simulink model "all_at_0001_0101"  (R2026a)
settings: Solver=ode5  StopTime=30  FixedStep=.01  AbsTol=1e-6
model workspace (MATLAB code in the model file):
  | load sldemo_autotrans_data; %load initial conditions and other necessary data
undefined symbols (not defined in the file): converter_data, downtab, emap, Iei, uptab, vehicledata
Description:
  | Modeling an Automatic Transmission Controller
  | 
  | In this example, Simulink(R) is used to model an automotive drivetrain. Stateflow(R)
  | enhances the Simulink model with its representation of the transmission
  | control logic. Simulink provides a powerful environment for the modeling and
  | simulation of dynamic systems and processes. In many systems, though,
  | supervisory functions like changing modes or invoking new gain schedules must
  | respond to events that may occur and conditions that develop over time. As a
  | result, the environment requires a language capable of managing these multiple
  | modes and developing conditions. In the following example, Stateflow
  | demonstrates its strength in this capacity by performing the function of gear
  | selection in an automatic transmission. This function is combined with the
  | drivetrain dynamics in a natural and intuitive manner by incorporating a
  | Stateflow block in the Simulink block diagram.
settings Model: DataTypeOverride=Double  MinMaxOverflowLogging=ForceOff  SimulationMode=accelerator  ExtModeTrigMode=oneshot  ExtModeArmWhenConnect=off  ExtModeAutoUpdateStatusClock=off  Creator=The MathWorks Inc.  LastModifiedBy=harry_31916
settings DataIOCC: ExternalInput=[t__, u__]  SignalLoggingName=sldemo_autotrans_output
settings OptimizationCC: BooleanDataType=off  InitFltsAndDblsToZero=on
settings DebuggingCC: SaveWithParameterizedLinksMsg=none  UnderspecifiedInitializationDetection=Classic  CheckExecutionContextPreStartOutputMsg=on  SignalResolutionControl=TryResolveAllWithWarning  MultiTaskDSMMsg=warning  MultiTaskCondExecSysMsg=none  SigSpecEnsureSampleTimeMsg=none  IntegerOverflowMsg=none  IntegerSaturationMsg=none
settings HardwareCC: ProdHWDeviceType=32-bit Generic
settings SFSimCC: SFSimEcho=off
settings GRTTargetCC: TargetFcnLib=ansi_tfl_tmw.mat  CombineOutputUpdateFcns=off  GRTInterface=on
settings ConfigComp: CovMetricSettings=dcmtr

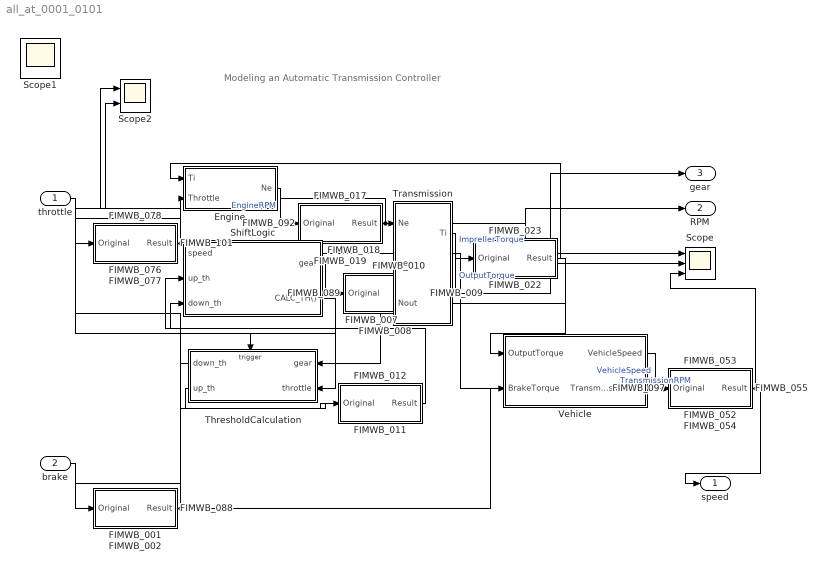
== system all_at_0001_0101 ==
  note: Modeling an Automatic Transmission Controller
  throttle : Inport  Interpolate=off
  brake : Inport  Port=2  Interpolate=off
  Engine : Subsystem
  FIMWB_001 : Subsystem  Tag=fimwb.fault.1
  FIMWB_002 : Subsystem  Tag=fimwb.fault.2
  FIMWB_007 : Subsystem  Tag=fimwb.fault.7
  FIMWB_008 : Subsystem  Tag=fimwb.fault.8
  FIMWB_009 : Subsystem  Tag=fimwb.fault.9
  FIMWB_010 : Subsystem  Tag=fimwb.fault.10
  FIMWB_011 : Subsystem  Tag=fimwb.fault.11
  FIMWB_012 : Subsystem  Tag=fimwb.fault.12
  FIMWB_017 : Subsystem  Tag=fimwb.fault.17
  FIMWB_018 : Subsystem  Tag=fimwb.fault.18
  FIMWB_019 : Subsystem  Tag=fimwb.fault.19
  FIMWB_022 : Subsystem  Tag=fimwb.fault.22
  FIMWB_023 : Subsystem  Tag=fimwb.fault.23
  FIMWB_052 : Subsystem  Tag=fimwb.fault.52
  FIMWB_053 : Subsystem  Tag=fimwb.fault.53
  FIMWB_054 : Subsystem  Tag=fimwb.fault.54
  FIMWB_055 : Subsystem  Tag=fimwb.fault.55
  FIMWB_076 : Subsystem  Tag=fimwb.fault.76
  FIMWB_077 : Subsystem  Tag=fimwb.fault.77
  FIMWB_078 : Subsystem  Tag=fimwb.fault.78
  FIMWB_088 : Subsystem  Tag=fimwb.fault.88
  FIMWB_089 : Subsystem  Tag=fimwb.fault.89
  FIMWB_092 : Subsystem  Tag=fimwb.fault.92
  FIMWB_097 : Subsystem  Tag=fimwb.fault.97
  FIMWB_101 : Subsystem  Tag=fimwb.fault.101
  Scope : Scope  NumInputPorts=3
      settings: ActiveDisplayYMinimum=-5  ActiveDisplayYMaximum=5
  Scope2 : Scope  NumInputPorts=2
      settings: ActiveDisplayYMinimum=-5  ActiveDisplayYMaximum=100
  ShiftLogic : Stateflow chart  TreatAsAtomicUnit=on
  ThresholdCalculation : Subsystem  TreatAsAtomicUnit=on
  Transmission : Subsystem
  Vehicle : Subsystem  mask(vehicle model){Rfd=vehicledata(1), rload0=vehicledata(2), rload2=vehicledata(3), Rw=vehicledata(4), Iv=vehicledata(5), N20=vehicledata(6)/vehicledata(4)*vehicledata(1)}
      mask prompts: Rfd "final drive ratio"; rload0 "drag friction at wheels"; rload2 "aerodynamic drag"; Rw "wheel radius"; Iv "vehicle inertia"; N20 "initial transmission output speed"
      mask help: vehicle dynamics: torque input from trans., outputs are input speed (transmission output) and vehicle speed
      mask Display: image(imread([matlabroot,'/toolbox/simulink/simdemos/automotive/html/NSX_3Colors.jpg']))
  speed : Outport  VectorParamsAs1DForOutWhenUnconnected=off
  RPM : Outport  Port=2  VectorParamsAs1DForOutWhenUnconnected=off
  gear : Outport  Port=3  VectorParamsAs1DForOutWhenUnconnected=off
  Scope1 : Scope
      settings: TimeSpan=30  ActiveDisplayYMinimum=1000  ActiveDisplayYMaximum=5000  DataLoggingMaxPoints=7500  DataLoggingSaveFormat=Array
  wires:
  ShiftLogic/2(CALC_TH()) -> ThresholdCalculation/Trigger
  brake/1 -> FIMWB_088/1(Original)
  FIMWB_088/1(Result) -> FIMWB_001/1(Original), FIMWB_002/1(Original)
  ShiftLogic/1(gear) -> FIMWB_089/1(Original)
  FIMWB_089/1(Result) -> FIMWB_007/1(Original), FIMWB_008/1(Original), FIMWB_009/1(Original), FIMWB_010/1(Original)
  Engine/1(Ne) -> FIMWB_092/1(Original)  "EngineRPM"
  FIMWB_092/1(Result) -> FIMWB_017/1(Original), FIMWB_018/1(Original), FIMWB_019/1(Original)
  Vehicle/1(VehicleSpeed) -> FIMWB_097/1(Original)  "VehicleSpeed"
  FIMWB_097/1(Result) -> FIMWB_052/1(Original), FIMWB_053/1(Original), FIMWB_054/1(Original)
  throttle/1 -> FIMWB_101/1(Original)
  FIMWB_101/1(Result) -> FIMWB_076/1(Original), FIMWB_077/1(Original), FIMWB_078/1(Original)
  FIMWB_001/1(Result) -> Scope2/2
  FIMWB_002/1(Result) -> Vehicle/2(BrakeTorque)
  FIMWB_007/1(Result) -> gear/1
  FIMWB_008/1(Result) -> Scope/1
  FIMWB_009/1(Result) -> ThresholdCalculation/1(gear)
  FIMWB_010/1(Result) -> Transmission/2(gear)
  ThresholdCalculation/1(down_th) -> FIMWB_011/1(Original)
  FIMWB_011/1(Result) -> ShiftLogic/3(down_th)
  ThresholdCalculation/2(up_th) -> FIMWB_012/1(Original)
  FIMWB_012/1(Result) -> ShiftLogic/2(up_th)
  FIMWB_017/1(Result) -> Scope/2
  FIMWB_018/1(Result) -> Transmission/1(Ne)
  FIMWB_019/1(Result) -> RPM/1
  Transmission/1(Ti) -> FIMWB_022/1(Original)  "ImprellerTorque"
  FIMWB_022/1(Result) -> Engine/1(Ti)
  Transmission/2(Tout) -> FIMWB_023/1(Original)  "OutputTorque"
  FIMWB_023/1(Result) -> Vehicle/1(OutputTorque)
  FIMWB_052/1(Result) -> Scope/3
  FIMWB_053/1(Result) -> ShiftLogic/1(speed)
  FIMWB_054/1(Result) -> speed/1
  Vehicle/2(TransmissionRPM) -> FIMWB_055/1(Original)  "TransmissionRPM"
  FIMWB_055/1(Result) -> Transmission/3(Nout)
  FIMWB_076/1(Result) -> Scope2/1
  FIMWB_077/1(Result) -> ThresholdCalculation/2(throttle)
  FIMWB_078/1(Result) -> Engine/2(Throttle)

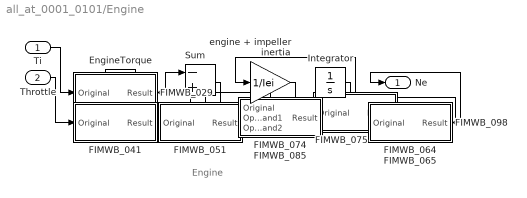
== system all_at_0001_0101/Engine ==
  note: Engine
  Ti : Inport
  Throttle : Inport  Port=2
  EngineTorque : Lookup2D  RowIndex=thvec  ColumnIndex=nevec  Table=emap  SaturateOnIntegerOverflow=off
  FIMWB_029 : Subsystem  Tag=fimwb.fault.29
  FIMWB_041 : Subsystem  Tag=fimwb.fault.41
  FIMWB_051 : Subsystem  Tag=fimwb.fault.51
  FIMWB_064 : Subsystem  Tag=fimwb.fault.64
  FIMWB_065 : Subsystem  Tag=fimwb.fault.65
  FIMWB_074 : Subsystem  Tag=fimwb.fault.74
  FIMWB_075 : Subsystem  Tag=fimwb.fault.75
  FIMWB_085 : Subsystem  Tag=fimwb.fault.85
  FIMWB_098 : Subsystem  Tag=fimwb.fault.98
  Integrator : Integrator  InitialCondition=1000  LimitOutput=on  UpperSaturationLimit=6000  LowerSaturationLimit=600  ZeroCross=off
  Sum : Sum  Inputs=-+  InputSameDT=on  SaturateOnIntegerOverflow=on  OutDataTypeStr=Inherit: Same as first input
  engine + impeller inertia : Gain  Gain=1/Iei  SaturateOnIntegerOverflow=on  OutDataTypeStr=Inherit: Same as input  ParamDataTypeStr=Inherit: Same as input
  Ne : Outport  InitialOutput=0  VectorParamsAs1DForOutWhenUnconnected=off
  wires:
  Sum/1 -> FIMWB_085/1(Original)
  Integrator/1 -> FIMWB_098/1(Original)
  FIMWB_098/1(Result) -> FIMWB_064/1(Original), FIMWB_065/1(Original)
  Ti/1 -> FIMWB_029/1(Original)
  FIMWB_029/1(Result) -> Sum/1, FIMWB_085/2(Operand1)
  Throttle/1 -> FIMWB_041/1(Original)
  FIMWB_041/1(Result) -> EngineTorque/1
  EngineTorque/1 -> FIMWB_051/1(Original)
  FIMWB_051/1(Result) -> Sum/2, FIMWB_085/3(Operand2)
  FIMWB_064/1(Result) -> EngineTorque/2
  FIMWB_065/1(Result) -> Ne/1
  FIMWB_085/1(Result) -> FIMWB_074/1(Original)
  FIMWB_074/1(Result) -> engine + impeller inertia/1
  engine + impeller inertia/1 -> FIMWB_075/1(Original)
  FIMWB_075/1(Result) -> Integrator/1

== system all_at_0001_0101/FIMWB_001 ==
  Original : Inport
  Result : Outport
  wires:
  Original/1 -> Result/1

== system all_at_0001_0101/FIMWB_002 ==
  Original : Inport
  Result : Outport
  wires:
  Original/1 -> Result/1

== system all_at_0001_0101/FIMWB_007 ==
  Original : Inport
  Result : Outport
  wires:
  Original/1 -> Result/1

== system all_at_0001_0101/FIMWB_008 ==
  Original : Inport
  Result : Outport
  wires:
  Original/1 -> Result/1

== system all_at_0001_0101/FIMWB_009 ==
  Original : Inport
  Result : Outport
  wires:
  Original/1 -> Result/1

== system all_at_0001_0101/FIMWB_010 ==
  Original : Inport
  Result : Outport
  wires:
  Original/1 -> Result/1

== system all_at_0001_0101/FIMWB_011 ==
  Original : Inport
  Result : Outport
  wires:
  Original/1 -> Result/1

== system all_at_0001_0101/FIMWB_012 ==
  Original : Inport
  Result : Outport
  wires:
  Original/1 -> Result/1

== system all_at_0001_0101/FIMWB_017 ==
  Original : Inport
  Result : Outport
  wires:
  Original/1 -> Result/1

== system all_at_0001_0101/FIMWB_018 ==
  Original : Inport
  Result : Outport
  wires:
  Original/1 -> Result/1

== system all_at_0001_0101/FIMWB_019 ==
  Original : Inport
  Result : Outport
  wires:
  Original/1 -> Result/1

== system all_at_0001_0101/FIMWB_022 ==
  Original : Inport
  Result : Outport
  wires:
  Original/1 -> Result/1

== system all_at_0001_0101/FIMWB_023 ==
  Original : Inport
  Result : Outport
  wires:
  Original/1 -> Result/1

== system all_at_0001_0101/FIMWB_052 ==
  Original : Inport
  Result : Outport
  wires:
  Original/1 -> Result/1

== system all_at_0001_0101/FIMWB_053 ==
  Original : Inport
  Result : Outport
  wires:
  Original/1 -> Result/1

== system all_at_0001_0101/FIMWB_054 ==
  Original : Inport
  Result : Outport
  wires:
  Original/1 -> Result/1

== system all_at_0001_0101/FIMWB_055 ==
  Original : Inport
  Result : Outport
  wires:
  Original/1 -> Result/1

== system all_at_0001_0101/FIMWB_076 ==
  Original : Inport
  Result : Outport
  wires:
  Original/1 -> Result/1

== system all_at_0001_0101/FIMWB_077 ==
  Original : Inport
  Result : Outport
  wires:
  Original/1 -> Result/1

== system all_at_0001_0101/FIMWB_078 ==
  Original : Inport
  Result : Outport
  wires:
  Original/1 -> Result/1

== system all_at_0001_0101/FIMWB_088 ==
  Original : Inport
  Result : Outport
  wires:
  Original/1 -> Result/1

== system all_at_0001_0101/FIMWB_089 ==
  Original : Inport
  Result : Outport
  wires:
  Original/1 -> Result/1

== system all_at_0001_0101/FIMWB_092 ==
  Original : Inport
  Result : Outport
  wires:
  Original/1 -> Result/1

== system all_at_0001_0101/FIMWB_097 ==
  Original : Inport
  Result : Outport
  wires:
  Original/1 -> Result/1

== system all_at_0001_0101/FIMWB_101 ==
  Original : Inport
  Result : Outport
  wires:
  Original/1 -> Result/1

== system all_at_0001_0101/ShiftLogic/FIMWB_003 ==
  Original : Inport
  Result : Outport
  wires:
  Original/1 -> Result/1

== system all_at_0001_0101/ShiftLogic/FIMWB_004 ==
  Original : Inport
  Result : Outport
  wires:
  Original/1 -> Result/1

== system all_at_0001_0101/ShiftLogic/FIMWB_005 ==
  Original : Inport
  Result : Outport
  wires:
  Original/1 -> Result/1

== system all_at_0001_0101/ShiftLogic/FIMWB_006 ==
  Original : Inport
  Result : Outport
  wires:
  Original/1 -> Result/1

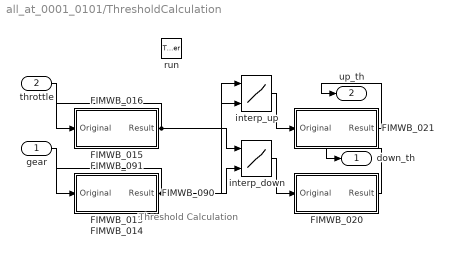
== system all_at_0001_0101/ThresholdCalculation ==
  note: Threshold Calculation
  gear : Inport
  throttle : Inport  Port=2
  run : TriggerPort  TriggerType=function-call  VariantControl=(inherit)  ZeroCross=off
  FIMWB_013 : Subsystem  Tag=fimwb.fault.13
  FIMWB_014 : Subsystem  Tag=fimwb.fault.14
  FIMWB_015 : Subsystem  Tag=fimwb.fault.15
  FIMWB_016 : Subsystem  Tag=fimwb.fault.16
  FIMWB_020 : Subsystem  Tag=fimwb.fault.20
  FIMWB_021 : Subsystem  Tag=fimwb.fault.21
  FIMWB_090 : Subsystem  Tag=fimwb.fault.90
  FIMWB_091 : Subsystem  Tag=fimwb.fault.91
  interp_down : Lookup2D  RowIndex=downth  ColumnIndex=[1:4]  Table=downtab  OutDataTypeStr=double  SaturateOnIntegerOverflow=off  InputSameDT=off
      settings: LockScale=on
  interp_up : Lookup2D  RowIndex=upth  ColumnIndex=[1:4]  Table=uptab  OutDataTypeStr=double  SaturateOnIntegerOverflow=off  InputSameDT=off
      settings: LockScale=on
  down_th : Outport  VectorParamsAs1DForOutWhenUnconnected=off
  up_th : Outport  Port=2  VectorParamsAs1DForOutWhenUnconnected=off
  wires:
  gear/1 -> FIMWB_090/1(Original)
  FIMWB_090/1(Result) -> FIMWB_013/1(Original), FIMWB_014/1(Original)
  throttle/1 -> FIMWB_091/1(Original)
  FIMWB_091/1(Result) -> FIMWB_015/1(Original), FIMWB_016/1(Original)
  FIMWB_013/1(Result) -> interp_down/2
  FIMWB_014/1(Result) -> interp_up/2
  FIMWB_015/1(Result) -> interp_down/1
  FIMWB_016/1(Result) -> interp_up/1
  interp_down/1 -> FIMWB_020/1(Original)
  FIMWB_020/1(Result) -> down_th/1
  interp_up/1 -> FIMWB_021/1(Original)
  FIMWB_021/1(Result) -> up_th/1

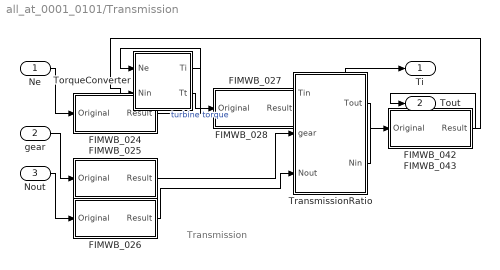
== system all_at_0001_0101/Transmission ==
  note: Transmission
  Ne : Inport
  gear : Inport  Port=2
  Nout : Inport  Port=3
  FIMWB_024 : Subsystem  Tag=fimwb.fault.24
  FIMWB_025 : Subsystem  Tag=fimwb.fault.25
  FIMWB_026 : Subsystem  Tag=fimwb.fault.26
  FIMWB_027 : Subsystem  Tag=fimwb.fault.27
  FIMWB_028 : Subsystem  Tag=fimwb.fault.28
  FIMWB_042 : Subsystem  Tag=fimwb.fault.42
  FIMWB_043 : Subsystem  Tag=fimwb.fault.43
  TorqueConverter : Subsystem  mask(torque converter){speedratio=converter_data(:,1), Kfactor=converter_data(:,2), Torkratio=converter_data(:,3)}
      mask prompts: speedratio "speed ratio"; Kfactor "K factor"; Torkratio "torque ratio"
      mask help: torque converter
      mask Help: Torque converter input and output torques are computed as a function of the input and output speeds
      mask Display: plot([cos([90:10:450]*pi/180),.63*cos([90:10:450]*pi/180),.63*cos([90:10:240]*pi/180),cos([240:10:300]*pi/180),.63*cos([300]*pi/180)],[sin([90:10:450]*pi/180),.63*sin([90:10:450]*pi/180)+.1,.63*sin([90:10:240]*pi/180)+.1,sin([240:10:300]*pi/180),.63*sin([300]*pi/180)+.1])
  TransmissionRatio : Subsystem
  Ti : Outport  InitialOutput=0  VectorParamsAs1DForOutWhenUnconnected=off
  Tout : Outport  Port=2  InitialOutput=0  VectorParamsAs1DForOutWhenUnconnected=off
  wires:
  Ne/1 -> FIMWB_024/1(Original)
  FIMWB_024/1(Result) -> TorqueConverter/1(Ne)
  gear/1 -> FIMWB_025/1(Original)
  FIMWB_025/1(Result) -> TransmissionRatio/2(gear)
  Nout/1 -> FIMWB_026/1(Original)
  FIMWB_026/1(Result) -> TransmissionRatio/3(Nout)
  TorqueConverter/1(Ti) -> FIMWB_027/1(Original)
  FIMWB_027/1(Result) -> Ti/1
  TorqueConverter/2(Tt) -> FIMWB_028/1(Original)  "turbine torque"
  FIMWB_028/1(Result) -> TransmissionRatio/1(Tin)
  TransmissionRatio/1(Tout) -> FIMWB_042/1(Original)
  FIMWB_042/1(Result) -> Tout/1
  TransmissionRatio/2(Nin) -> FIMWB_043/1(Original)
  FIMWB_043/1(Result) -> TorqueConverter/2(Nin)

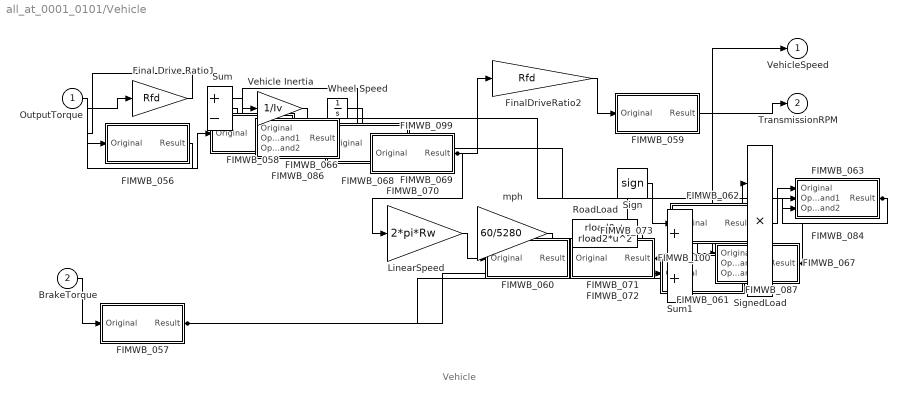
== system all_at_0001_0101/Vehicle ==
  note: Vehicle
  OutputTorque : Inport
  BrakeTorque : Inport  Port=2
  FIMWB_056 : Subsystem  Tag=fimwb.fault.56
  FIMWB_057 : Subsystem  Tag=fimwb.fault.57
  FIMWB_058 : Subsystem  Tag=fimwb.fault.58
  FIMWB_059 : Subsystem  Tag=fimwb.fault.59
  FIMWB_060 : Subsystem  Tag=fimwb.fault.60
  FIMWB_061 : Subsystem  Tag=fimwb.fault.61
  FIMWB_062 : Subsystem  Tag=fimwb.fault.62
  FIMWB_063 : Subsystem  Tag=fimwb.fault.63
  FIMWB_066 : Subsystem  Tag=fimwb.fault.66
  FIMWB_067 : Subsystem  Tag=fimwb.fault.67
  FIMWB_068 : Subsystem  Tag=fimwb.fault.68
  FIMWB_069 : Subsystem  Tag=fimwb.fault.69
  FIMWB_070 : Subsystem  Tag=fimwb.fault.70
  FIMWB_071 : Subsystem  Tag=fimwb.fault.71
  FIMWB_072 : Subsystem  Tag=fimwb.fault.72
  FIMWB_073 : Subsystem  Tag=fimwb.fault.73
  FIMWB_084 : Subsystem  Tag=fimwb.fault.84
  FIMWB_086 : Subsystem  Tag=fimwb.fault.86
  FIMWB_087 : Subsystem  Tag=fimwb.fault.87
  FIMWB_099 : Subsystem  Tag=fimwb.fault.99
  FIMWB_100 : Subsystem  Tag=fimwb.fault.100
  Final Drive Ratio1 : Gain  Gain=Rfd  SaturateOnIntegerOverflow=on  OutDataTypeStr=Inherit: Same as input  ParamDataTypeStr=Inherit: Same as input
  FinalDriveRatio2 : Gain  Gain=Rfd  SaturateOnIntegerOverflow=on  OutDataTypeStr=Inherit: Same as input  ParamDataTypeStr=Inherit: Same as input
  LinearSpeed : Gain  Gain=2*pi*Rw  SaturateOnIntegerOverflow=on  OutDataTypeStr=Inherit: Same as input  ParamDataTypeStr=Inherit: Same as input
  RoadLoad : Fcn  Expr=rload0 + rload2*u^2
  Sign : Signum
  SignedLoad : Product  InputSameDT=on  SaturateOnIntegerOverflow=on  OutDataTypeStr=Inherit: Same as first input
  Sum : Sum  Inputs=+-  InputSameDT=on  SaturateOnIntegerOverflow=on  OutDataTypeStr=Inherit: Same as first input
  Sum1 : Sum  InputSameDT=on  SaturateOnIntegerOverflow=on  OutDataTypeStr=Inherit: Same as first input
  Vehicle Inertia : Gain  Gain=1/Iv  SaturateOnIntegerOverflow=on  OutDataTypeStr=Inherit: Same as input  ParamDataTypeStr=Inherit: Same as input
  Wheel Speed : Integrator  InitialCondition=N20/Rfd  ZeroCross=off
  mph : Gain  Gain=60/5280  SaturateOnIntegerOverflow=on  OutDataTypeStr=Inherit: Same as input  ParamDataTypeStr=Inherit: Same as input
  VehicleSpeed : Outport  InitialOutput=0  VectorParamsAs1DForOutWhenUnconnected=off
  TransmissionRPM : Outport  Port=2  InitialOutput=0  VectorParamsAs1DForOutWhenUnconnected=off
  wires:
  SignedLoad/1 -> FIMWB_084/1(Original)
  Sum/1 -> FIMWB_086/1(Original)
  Sum1/1 -> FIMWB_087/1(Original)
  Wheel Speed/1 -> FIMWB_099/1(Original)
  FIMWB_099/1(Result) -> FIMWB_069/1(Original), FIMWB_070/1(Original)
  mph/1 -> FIMWB_100/1(Original)
  FIMWB_100/1(Result) -> FIMWB_071/1(Original), FIMWB_072/1(Original), FIMWB_073/1(Original)
  OutputTorque/1 -> FIMWB_056/1(Original)
  FIMWB_056/1(Result) -> Final Drive Ratio1/1
  BrakeTorque/1 -> FIMWB_057/1(Original)
  FIMWB_057/1(Result) -> Sum1/2, FIMWB_087/3(Operand2)
  Final Drive Ratio1/1 -> FIMWB_058/1(Original)
  FIMWB_058/1(Result) -> Sum/1, FIMWB_086/2(Operand1)
  FinalDriveRatio2/1 -> FIMWB_059/1(Original)
  FIMWB_059/1(Result) -> TransmissionRPM/1
  LinearSpeed/1 -> FIMWB_060/1(Original)
  FIMWB_060/1(Result) -> mph/1
  RoadLoad/1 -> FIMWB_061/1(Original)
  FIMWB_061/1(Result) -> Sum1/1, FIMWB_087/2(Operand1)
  Sign/1 -> FIMWB_062/1(Original)
  FIMWB_062/1(Result) -> SignedLoad/1, FIMWB_084/2(Operand1)
  FIMWB_084/1(Result) -> FIMWB_063/1(Original)
  FIMWB_063/1(Result) -> Sum/2, FIMWB_086/3(Operand2)
  FIMWB_086/1(Result) -> FIMWB_066/1(Original)
  FIMWB_066/1(Result) -> Vehicle Inertia/1
  FIMWB_087/1(Result) -> FIMWB_067/1(Original)
  FIMWB_067/1(Result) -> SignedLoad/2, FIMWB_084/3(Operand2)
  Vehicle Inertia/1 -> FIMWB_068/1(Original)
  FIMWB_068/1(Result) -> Wheel Speed/1
  FIMWB_069/1(Result) -> FinalDriveRatio2/1
  FIMWB_070/1(Result) -> LinearSpeed/1
  FIMWB_071/1(Result) -> RoadLoad/1
  FIMWB_072/1(Result) -> Sign/1
  FIMWB_073/1(Result) -> VehicleSpeed/1

== system all_at_0001_0101/Engine/FIMWB_029 ==
  Original : Inport
  Result : Outport
  wires:
  Original/1 -> Result/1

== system all_at_0001_0101/Engine/FIMWB_041 ==
  Original : Inport
  Result : Outport
  wires:
  Original/1 -> Result/1

== system all_at_0001_0101/Engine/FIMWB_051 ==
  Original : Inport
  Result : Outport
  wires:
  Original/1 -> Result/1

== system all_at_0001_0101/Engine/FIMWB_064 ==
  Original : Inport
  Result : Outport
  wires:
  Original/1 -> Result/1

== system all_at_0001_0101/Engine/FIMWB_065 ==
  Original : Inport
  Result : Outport
  wires:
  Original/1 -> Result/1

== system all_at_0001_0101/Engine/FIMWB_074 ==
  Original : Inport
  Result : Outport
  wires:
  Original/1 -> Result/1

== system all_at_0001_0101/Engine/FIMWB_075 ==
  Original : Inport
  Result : Outport
  wires:
  Original/1 -> Result/1

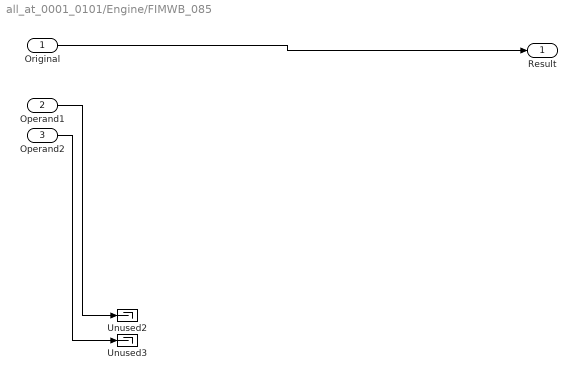
== system all_at_0001_0101/Engine/FIMWB_085 ==
  Original : Inport
  Operand1 : Inport  Port=2
  Operand2 : Inport  Port=3
  Unused2 : Terminator
  Unused3 : Terminator
  Result : Outport
  wires:
  Original/1 -> Result/1
  Operand1/1 -> Unused2/1
  Operand2/1 -> Unused3/1

== system all_at_0001_0101/Engine/FIMWB_098 ==
  Original : Inport
  Result : Outport
  wires:
  Original/1 -> Result/1

== system all_at_0001_0101/ThresholdCalculation/FIMWB_013 ==
  Original : Inport
  Result : Outport
  wires:
  Original/1 -> Result/1

== system all_at_0001_0101/ThresholdCalculation/FIMWB_014 ==
  Original : Inport
  Result : Outport
  wires:
  Original/1 -> Result/1

== system all_at_0001_0101/ThresholdCalculation/FIMWB_015 ==
  Original : Inport
  Result : Outport
  wires:
  Original/1 -> Result/1

== system all_at_0001_0101/ThresholdCalculation/FIMWB_016 ==
  Original : Inport
  Result : Outport
  wires:
  Original/1 -> Result/1

== system all_at_0001_0101/ThresholdCalculation/FIMWB_020 ==
  Original : Inport
  Result : Outport
  wires:
  Original/1 -> Result/1

== system all_at_0001_0101/ThresholdCalculation/FIMWB_021 ==
  Original : Inport
  Result : Outport
  wires:
  Original/1 -> Result/1

== system all_at_0001_0101/ThresholdCalculation/FIMWB_090 ==
  Original : Inport
  Result : Outport
  wires:
  Original/1 -> Result/1

== system all_at_0001_0101/ThresholdCalculation/FIMWB_091 ==
  Original : Inport
  Result : Outport
  wires:
  Original/1 -> Result/1

== system all_at_0001_0101/Transmission/FIMWB_024 ==
  Original : Inport
  Result : Outport
  wires:
  Original/1 -> Result/1

== system all_at_0001_0101/Transmission/FIMWB_025 ==
  Original : Inport
  Result : Outport
  wires:
  Original/1 -> Result/1

== system all_at_0001_0101/Transmission/FIMWB_026 ==
  Original : Inport
  Result : Outport
  wires:
  Original/1 -> Result/1

== system all_at_0001_0101/Transmission/FIMWB_027 ==
  Original : Inport
  Result : Outport
  wires:
  Original/1 -> Result/1

== system all_at_0001_0101/Transmission/FIMWB_028 ==
  Original : Inport
  Result : Outport
  wires:
  Original/1 -> Result/1

== system all_at_0001_0101/Transmission/FIMWB_042 ==
  Original : Inport
  Result : Outport
  wires:
  Original/1 -> Result/1

== system all_at_0001_0101/Transmission/FIMWB_043 ==
  Original : Inport
  Result : Outport
  wires:
  Original/1 -> Result/1

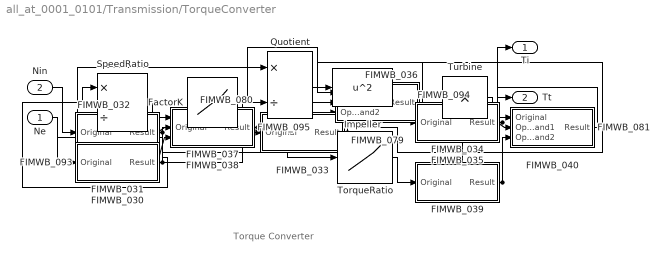
== system all_at_0001_0101/Transmission/TorqueConverter ==
  note: Torque Converter
  Ne : Inport
  Nin : Inport  Port=2
  FIMWB_030 : Subsystem  Tag=fimwb.fault.30
  FIMWB_031 : Subsystem  Tag=fimwb.fault.31
  FIMWB_032 : Subsystem  Tag=fimwb.fault.32
  FIMWB_033 : Subsystem  Tag=fimwb.fault.33
  FIMWB_034 : Subsystem  Tag=fimwb.fault.34
  FIMWB_035 : Subsystem  Tag=fimwb.fault.35
  FIMWB_036 : Subsystem  Tag=fimwb.fault.36
  FIMWB_037 : Subsystem  Tag=fimwb.fault.37
  FIMWB_038 : Subsystem  Tag=fimwb.fault.38
  FIMWB_039 : Subsystem  Tag=fimwb.fault.39
  FIMWB_040 : Subsystem  Tag=fimwb.fault.40
  FIMWB_079 : Subsystem  Tag=fimwb.fault.79
  FIMWB_080 : Subsystem  Tag=fimwb.fault.80
  FIMWB_081 : Subsystem  Tag=fimwb.fault.81
  FIMWB_093 : Subsystem  Tag=fimwb.fault.93
  FIMWB_094 : Subsystem  Tag=fimwb.fault.94
  FIMWB_095 : Subsystem  Tag=fimwb.fault.95
  FactorK : Lookup  InputValues=speedratio  Table=Kfactor
  Impeller : Fcn  Expr=u^2
  Quotient : Product  Inputs=*/  InputSameDT=on  SaturateOnIntegerOverflow=on  OutDataTypeStr=Inherit: Same as first input
  SpeedRatio : Product  Inputs=*/  InputSameDT=on  SaturateOnIntegerOverflow=on  OutDataTypeStr=Inherit: Same as first input
  TorqueRatio : Lookup  InputValues=speedratio  Table=Torkratio
  Turbine : Product  InputSameDT=on  SaturateOnIntegerOverflow=on  OutDataTypeStr=Inherit: Same as first input
  Ti : Outport  InitialOutput=0  VectorParamsAs1DForOutWhenUnconnected=off
  Tt : Outport  Port=2  InitialOutput=0  VectorParamsAs1DForOutWhenUnconnected=off
  wires:
  Quotient/1 -> FIMWB_079/1(Original)
  SpeedRatio/1 -> FIMWB_080/1(Original)
  Turbine/1 -> FIMWB_081/1(Original)
  Ne/1 -> FIMWB_093/1(Original)
  FIMWB_093/1(Result) -> FIMWB_030/1(Original), FIMWB_031/1(Original)
  Impeller/1 -> FIMWB_094/1(Original)
  FIMWB_094/1(Result) -> FIMWB_034/1(Original), FIMWB_035/1(Original)
  FIMWB_080/1(Result) -> FIMWB_095/1(Original)
  FIMWB_095/1(Result) -> FIMWB_037/1(Original), FIMWB_038/1(Original)
  FIMWB_030/1(Result) -> Quotient/1, FIMWB_079/2(Operand1)
  FIMWB_031/1(Result) -> SpeedRatio/2, FIMWB_080/3(Operand2)
  Nin/1 -> FIMWB_032/1(Original)
  FIMWB_032/1(Result) -> SpeedRatio/1, FIMWB_080/2(Operand1)
  FactorK/1 -> FIMWB_033/1(Original)
  FIMWB_033/1(Result) -> Quotient/2, FIMWB_079/3(Operand2)
  FIMWB_034/1(Result) -> Turbine/1, FIMWB_081/2(Operand1)
  FIMWB_035/1(Result) -> Ti/1
  FIMWB_079/1(Result) -> FIMWB_036/1(Original)
  FIMWB_036/1(Result) -> Impeller/1
  FIMWB_037/1(Result) -> FactorK/1
  FIMWB_038/1(Result) -> TorqueRatio/1
  TorqueRatio/1 -> FIMWB_039/1(Original)
  FIMWB_039/1(Result) -> Turbine/2, FIMWB_081/3(Operand2)
  FIMWB_081/1(Result) -> FIMWB_040/1(Original)
  FIMWB_040/1(Result) -> Tt/1

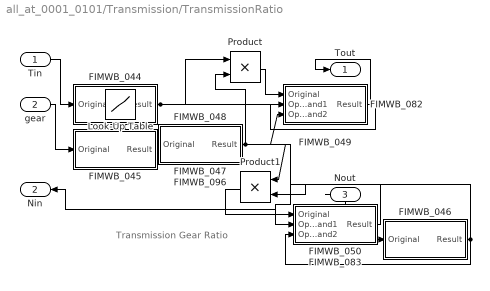
== system all_at_0001_0101/Transmission/TransmissionRatio ==
  note: Transmission Gear Ratio
  Tin : Inport
  gear : Inport  Port=2
  Nout : Inport  Port=3
  FIMWB_044 : Subsystem  Tag=fimwb.fault.44
  FIMWB_045 : Subsystem  Tag=fimwb.fault.45
  FIMWB_046 : Subsystem  Tag=fimwb.fault.46
  FIMWB_047 : Subsystem  Tag=fimwb.fault.47
  FIMWB_048 : Subsystem  Tag=fimwb.fault.48
  FIMWB_049 : Subsystem  Tag=fimwb.fault.49
  FIMWB_050 : Subsystem  Tag=fimwb.fault.50
  FIMWB_082 : Subsystem  Tag=fimwb.fault.82
  FIMWB_083 : Subsystem  Tag=fimwb.fault.83
  FIMWB_096 : Subsystem  Tag=fimwb.fault.96
  Look-Up Table : Lookup  InputValues=[1 2 3 4]  Table=[2.393 1.450 1.000 0.677]  OutDataTypeStr=double  LockScale=on
  Product : Product  InputSameDT=on  SaturateOnIntegerOverflow=on  OutDataTypeStr=Inherit: Same as first input
  Product1 : Product  InputSameDT=on  SaturateOnIntegerOverflow=on  OutDataTypeStr=Inherit: Same as first input
  Tout : Outport  InitialOutput=0  VectorParamsAs1DForOutWhenUnconnected=off
  Nin : Outport  Port=2  InitialOutput=0  VectorParamsAs1DForOutWhenUnconnected=off
  wires:
  Product/1 -> FIMWB_082/1(Original)
  Product1/1 -> FIMWB_083/1(Original)
  Look-Up Table/1 -> FIMWB_096/1(Original)
  FIMWB_096/1(Result) -> FIMWB_047/1(Original), FIMWB_048/1(Original)
  Tin/1 -> FIMWB_044/1(Original)
  FIMWB_044/1(Result) -> Product/1, FIMWB_082/2(Operand1)
  gear/1 -> FIMWB_045/1(Original)
  FIMWB_045/1(Result) -> Look-Up Table/1
  Nout/1 -> FIMWB_046/1(Original)
  FIMWB_046/1(Result) -> Product1/2, FIMWB_083/3(Operand2)
  FIMWB_047/1(Result) -> Product/2, FIMWB_082/3(Operand2)
  FIMWB_048/1(Result) -> Product1/1, FIMWB_083/2(Operand1)
  FIMWB_082/1(Result) -> FIMWB_049/1(Original)
  FIMWB_049/1(Result) -> Tout/1
  FIMWB_083/1(Result) -> FIMWB_050/1(Original)
  FIMWB_050/1(Result) -> Nin/1

== system all_at_0001_0101/Vehicle/FIMWB_056 ==
  Original : Inport
  Result : Outport
  wires:
  Original/1 -> Result/1

== system all_at_0001_0101/Vehicle/FIMWB_057 ==
  Original : Inport
  Result : Outport
  wires:
  Original/1 -> Result/1

== system all_at_0001_0101/Vehicle/FIMWB_058 ==
  Original : Inport
  Result : Outport
  wires:
  Original/1 -> Result/1

== system all_at_0001_0101/Vehicle/FIMWB_059 ==
  Original : Inport
  Result : Outport
  wires:
  Original/1 -> Result/1

== system all_at_0001_0101/Vehicle/FIMWB_060 ==
  Original : Inport
  Result : Outport
  wires:
  Original/1 -> Result/1

== system all_at_0001_0101/Vehicle/FIMWB_061 ==
  Original : Inport
  Result : Outport
  wires:
  Original/1 -> Result/1

== system all_at_0001_0101/Vehicle/FIMWB_062 ==
  Original : Inport
  Result : Outport
  wires:
  Original/1 -> Result/1

== system all_at_0001_0101/Vehicle/FIMWB_063 ==
  Original : Inport
  Result : Outport
  wires:
  Original/1 -> Result/1

== system all_at_0001_0101/Vehicle/FIMWB_066 ==
  Original : Inport
  Result : Outport
  wires:
  Original/1 -> Result/1

== system all_at_0001_0101/Vehicle/FIMWB_067 ==
  Original : Inport
  Result : Outport
  wires:
  Original/1 -> Result/1

== system all_at_0001_0101/Vehicle/FIMWB_068 ==
  Original : Inport
  Result : Outport
  wires:
  Original/1 -> Result/1

== system all_at_0001_0101/Vehicle/FIMWB_069 ==
  Original : Inport
  Result : Outport
  wires:
  Original/1 -> Result/1

== system all_at_0001_0101/Vehicle/FIMWB_070 ==
  Original : Inport
  Result : Outport
  wires:
  Original/1 -> Result/1

== system all_at_0001_0101/Vehicle/FIMWB_071 ==
  Original : Inport
  Result : Outport
  wires:
  Original/1 -> Result/1

== system all_at_0001_0101/Vehicle/FIMWB_072 ==
  Original : Inport
  Result : Outport
  wires:
  Original/1 -> Result/1

== system all_at_0001_0101/Vehicle/FIMWB_073 ==
  Original : Inport
  Result : Outport
  wires:
  Original/1 -> Result/1

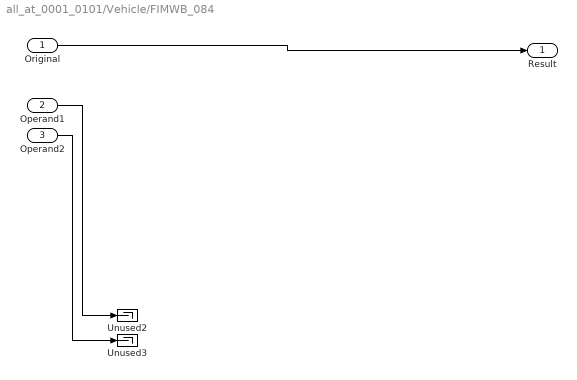
== system all_at_0001_0101/Vehicle/FIMWB_084 ==
  Original : Inport
  Operand1 : Inport  Port=2
  Operand2 : Inport  Port=3
  Unused2 : Terminator
  Unused3 : Terminator
  Result : Outport
  wires:
  Original/1 -> Result/1
  Operand1/1 -> Unused2/1
  Operand2/1 -> Unused3/1

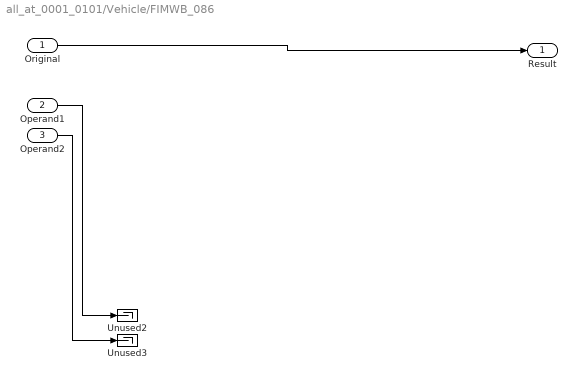
== system all_at_0001_0101/Vehicle/FIMWB_086 ==
  Original : Inport
  Operand1 : Inport  Port=2
  Operand2 : Inport  Port=3
  Unused2 : Terminator
  Unused3 : Terminator
  Result : Outport
  wires:
  Original/1 -> Result/1
  Operand1/1 -> Unused2/1
  Operand2/1 -> Unused3/1

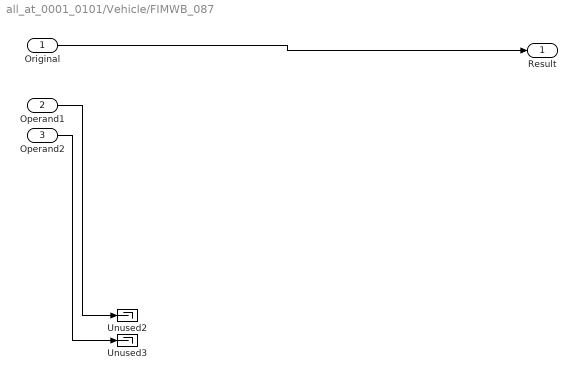
== system all_at_0001_0101/Vehicle/FIMWB_087 ==
  Original : Inport
  Operand1 : Inport  Port=2
  Operand2 : Inport  Port=3
  Unused2 : Terminator
  Unused3 : Terminator
  Result : Outport
  wires:
  Original/1 -> Result/1
  Operand1/1 -> Unused2/1
  Operand2/1 -> Unused3/1

== system all_at_0001_0101/Vehicle/FIMWB_099 ==
  Original : Inport
  Result : Outport
  wires:
  Original/1 -> Result/1

== system all_at_0001_0101/Vehicle/FIMWB_100 ==
  Original : Inport
  Result : Outport
  wires:
  Original/1 -> Result/1

== system all_at_0001_0101/Transmission/TorqueConverter/FIMWB_030 ==
  Original : Inport
  Result : Outport
  wires:
  Original/1 -> Result/1

== system all_at_0001_0101/Transmission/TorqueConverter/FIMWB_031 ==
  Original : Inport
  Result : Outport
  wires:
  Original/1 -> Result/1

== system all_at_0001_0101/Transmission/TorqueConverter/FIMWB_032 ==
  Original : Inport
  Result : Outport
  wires:
  Original/1 -> Result/1

== system all_at_0001_0101/Transmission/TorqueConverter/FIMWB_033 ==
  Original : Inport
  Result : Outport
  wires:
  Original/1 -> Result/1

== system all_at_0001_0101/Transmission/TorqueConverter/FIMWB_034 ==
  Original : Inport
  Result : Outport
  wires:
  Original/1 -> Result/1

== system all_at_0001_0101/Transmission/TorqueConverter/FIMWB_035 ==
  Original : Inport
  Result : Outport
  wires:
  Original/1 -> Result/1

== system all_at_0001_0101/Transmission/TorqueConverter/FIMWB_036 ==
  Original : Inport
  Result : Outport
  wires:
  Original/1 -> Result/1

== system all_at_0001_0101/Transmission/TorqueConverter/FIMWB_037 ==
  Original : Inport
  Result : Outport
  wires:
  Original/1 -> Result/1

== system all_at_0001_0101/Transmission/TorqueConverter/FIMWB_038 ==
  Original : Inport
  Result : Outport
  wires:
  Original/1 -> Result/1

== system all_at_0001_0101/Transmission/TorqueConverter/FIMWB_039 ==
  Original : Inport
  Result : Outport
  wires:
  Original/1 -> Result/1

== system all_at_0001_0101/Transmission/TorqueConverter/FIMWB_040 ==
  Original : Inport
  Result : Outport
  wires:
  Original/1 -> Result/1

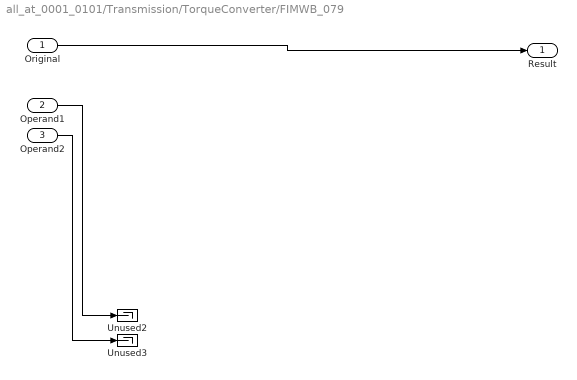
== system all_at_0001_0101/Transmission/TorqueConverter/FIMWB_079 ==
  Original : Inport
  Operand1 : Inport  Port=2
  Operand2 : Inport  Port=3
  Unused2 : Terminator
  Unused3 : Terminator
  Result : Outport
  wires:
  Original/1 -> Result/1
  Operand1/1 -> Unused2/1
  Operand2/1 -> Unused3/1

== system all_at_0001_0101/Transmission/TorqueConverter/FIMWB_080 ==
  Original : Inport
  Operand1 : Inport  Port=2
  Operand2 : Inport  Port=3
  Unused2 : Terminator
  Unused3 : Terminator
  Result : Outport
  wires:
  Original/1 -> Result/1
  Operand1/1 -> Unused2/1
  Operand2/1 -> Unused3/1

== system all_at_0001_0101/Transmission/TorqueConverter/FIMWB_081 ==
  Original : Inport
  Operand1 : Inport  Port=2
  Operand2 : Inport  Port=3
  Unused2 : Terminator
  Unused3 : Terminator
  Result : Outport
  wires:
  Original/1 -> Result/1
  Operand1/1 -> Unused2/1
  Operand2/1 -> Unused3/1

== system all_at_0001_0101/Transmission/TorqueConverter/FIMWB_093 ==
  Original : Inport
  Result : Outport
  wires:
  Original/1 -> Result/1

== system all_at_0001_0101/Transmission/TorqueConverter/FIMWB_094 ==
  Original : Inport
  Result : Outport
  wires:
  Original/1 -> Result/1

== system all_at_0001_0101/Transmission/TorqueConverter/FIMWB_095 ==
  Original : Inport
  Result : Outport
  wires:
  Original/1 -> Result/1

== system all_at_0001_0101/Transmission/TransmissionRatio/FIMWB_044 ==
  Original : Inport
  Result : Outport
  wires:
  Original/1 -> Result/1

== system all_at_0001_0101/Transmission/TransmissionRatio/FIMWB_045 ==
  Original : Inport
  Result : Outport
  wires:
  Original/1 -> Result/1

== system all_at_0001_0101/Transmission/TransmissionRatio/FIMWB_046 ==
  Original : Inport
  Result : Outport
  wires:
  Original/1 -> Result/1

== system all_at_0001_0101/Transmission/TransmissionRatio/FIMWB_047 ==
  Original : Inport
  Result : Outport
  wires:
  Original/1 -> Result/1

== system all_at_0001_0101/Transmission/TransmissionRatio/FIMWB_048 ==
  Original : Inport
  Result : Outport
  wires:
  Original/1 -> Result/1

== system all_at_0001_0101/Transmission/TransmissionRatio/FIMWB_049 ==
  Original : Inport
  Result : Outport
  wires:
  Original/1 -> Result/1

== system all_at_0001_0101/Transmission/TransmissionRatio/FIMWB_050 ==
  Original : Inport
  Result : Outport
  wires:
  Original/1 -> Result/1

== system all_at_0001_0101/Transmission/TransmissionRatio/FIMWB_082 ==
  Original : Inport
  Operand1 : Inport  Port=2
  Operand2 : Inport  Port=3
  Unused2 : Terminator
  Unused3 : Terminator
  Result : Outport
  wires:
  Original/1 -> Result/1
  Operand1/1 -> Unused2/1
  Operand2/1 -> Unused3/1

== system all_at_0001_0101/Transmission/TransmissionRatio/FIMWB_083 ==
  Original : Inport
  Operand1 : Inport  Port=2
  Operand2 : Inport  Port=3
  Unused2 : Terminator
  Unused3 : Terminator
  Result : Outport
  wires:
  Original/1 -> Result/1
  Operand1/1 -> Unused2/1
  Operand2/1 -> Unused3/1

== system all_at_0001_0101/Transmission/TransmissionRatio/FIMWB_096 ==
  Original : Inport
  Result : Outport
  wires:
  Original/1 -> Result/1

== stateflow chart all_at_0001_0101/ShiftLogic ==
  settings: updateMethod=DISCRETE  sampleTime=0.04
  state gear_state [parallel]
    settings: executionOrder=1
    state fourth
      entry:
      gear = 4;
    state third
      entry:
      gear = 3;
    state second
      entry:
      gear = 2;
    state first
      entry:
      gear = 1;
    (default) -> first
    second -> third [order 1] : UP
    first -> second : UP
    third -> fourth [order 1] : UP
    second -> first [order 2] : DOWN
    fourth -> third : DOWN
    third -> second [order 2] : DOWN
  state selection_state [parallel]
    during: CALC_TH;
    settings: executionOrder=2
    state steady_state
    state upshifting
    state downshifting
    (default) -> steady_state
    steady_state -> upshifting [order 1] : [speed > up_th]
    steady_state -> downshifting [order 2] : [speed < down_th]
    downshifting -> steady_state [order 1] : after(TWAIT,tick)
        | [speed <= down_th]
        | {gear_state.DOWN}
    downshifting -> steady_state [order 2] : [speed > down_th]
    upshifting -> steady_state [order 1] : after(TWAIT,tick)
        | [speed >= up_th]
        | {gear_state.UP}
    upshifting -> steady_state [order 2] : [speed < up_th]
  data: speed input double; gear output fixdt(0,8,5) [1..4]; TWAIT parameter fixdt(0,8,6); up_th input double; down_th input double
  events: DOWN local EITHER_EDGE_EVENT; UP local EITHER_EDGE_EVENT; CALC_TH output FUNCTION_CALL_EVENT
